simulink model "chaine_ham74"  (R2023b)
settings: Solver=FixedStepDiscrete  StartTime=0.0  StopTime=Nb*Tbi  FixedStep=1  RelTol=1e-3
undefined symbols (not defined in the file): a_c, dly, L, sig2, Tbi
settings Model: Creator=e2507457  LastModifiedBy=e2507457

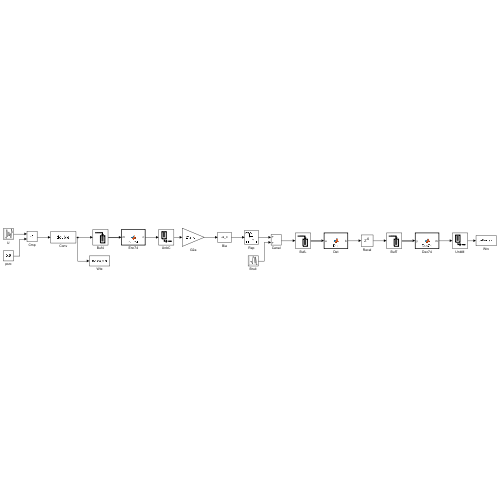
[thumbnail: Simulink's stored preview of the top-level diagram]
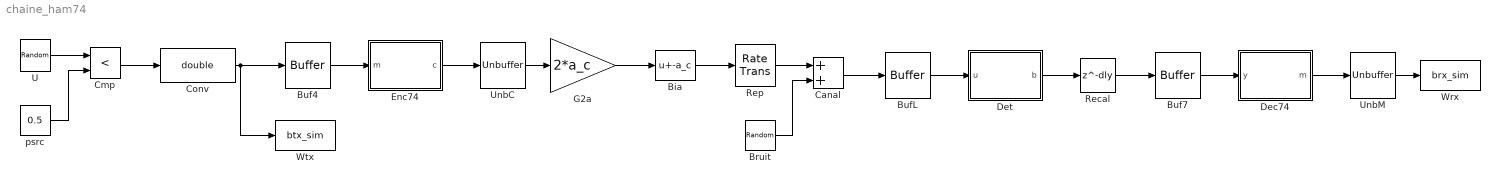
== system chaine_ham74 ==
  Bia : Bias  Bias=-a_c  SaturateOnIntegerOverflow=off
  Bruit : RandomNumber  Variance=sig2  Seed=32  SampleTime=1
  Buf4 : Buffer  N=4
  Buf7 : Buffer  N=7
  BufL : Buffer  N=L
  Canal : Sum
  Cmp : RelationalOperator  Operator=<  OutDataTypeStr=boolean  RndMeth=Simplest  InputSameDT=off
  Conv : DataTypeConversion  OutDataTypeStr=double  SaturateOnIntegerOverflow=off  RndMeth=Floor
  Dec74 : MATLAB Function  TreatAsAtomicUnit=on
  Det : MATLAB Function  TreatAsAtomicUnit=on
  Enc74 : MATLAB Function  TreatAsAtomicUnit=on
  G2a : Gain  Gain=2*a_c
  Recal : Delay  DelayLength=dly  InitialCondition=0  SampleTime=L
  Rep : RateTransition  Integrity=off  Deterministic=off  OutPortSampleTime=1
  U : UniformRandomNumber  Minimum=0  Seed=31  SampleTime=Tbi
  UnbC : Unbuffer
  UnbM : Unbuffer
  Wrx : ToWorkspace  VariableName=brx_sim  SampleTime=-1
  Wtx : ToWorkspace  VariableName=btx_sim  SampleTime=-1
  psrc : Constant  Value=0.5  SampleTime=Tbi
  wires:
  U/1 -> Cmp/1
  UnbC/1 -> G2a/1
  psrc/1 -> Cmp/2
  Cmp/1 -> Conv/1
  Enc74/1(c) -> UnbC/1
  Conv/1 -> Buf4/1, Wtx/1
  Buf4/1 -> Enc74/1(m)
  G2a/1 -> Bia/1
  Bia/1 -> Rep/1
  Rep/1 -> Canal/1
  Bruit/1 -> Canal/2
  Canal/1 -> BufL/1
  BufL/1 -> Det/1(u)
  Det/1(b) -> Recal/1
  Recal/1 -> Buf7/1
  Buf7/1 -> Dec74/1(y)
  Dec74/1(m) -> UnbM/1
  UnbM/1 -> Wrx/1

== matlab function chaine_ham74/Enc74 ==
  data: m input; c output
function c = Enc74(m)
%#codegen
c = [m(1); m(2); m(3); m(4); ...
     mod(m(1)+m(3)+m(4),2); ...
     mod(m(1)+m(2)+m(3),2); ...
     mod(m(2)+m(3)+m(4),2)];
end

== matlab function chaine_ham74/Dec74 ==
  data: y input; m output
function m = Dec74(y)
%#codegen
s0 = mod(y(1)+y(3)+y(4)+y(5), 2);
s1 = mod(y(1)+y(2)+y(3)+y(6), 2);
s2 = mod(y(2)+y(3)+y(4)+y(7), 2);
v  = 4*s0 + 2*s1 + s2;
m  = y(1:4);
if v == 6, m(1) = 1 - m(1); end
if v == 3, m(2) = 1 - m(2); end
if v == 7, m(3) = 1 - m(3); end
if v == 5, m(4) = 1 - m(4); end
end

== matlab function chaine_ham74/Det ==
  data: u input; b output
function b = Det(u)
%#codegen
b = double(mean(u(:)) > 0);
end
